simulink model "motor_maxon_EC20flat_351006"  (R2026a)
settings: Solver=FixedStepDiscrete  StopTime=5  FixedStep=Ts_sim
InitFcn:
  | warning('off','physmod:simscape:engine:core:advancer_errors:fallback_solve')
model workspace (MAT data in the model file):
  B_motor = 3.66016133122e-07
  B_rotor = 2e-07
  B_turntable = 5e-06
  C_buck = 4.7e-05
  Dmax = 0.95
  Fsw = 50000
  I_max = 1.5
  J_body = 0.002
  J_flywheel = 2.34905654183e-05
  J_rotor = 5.1e-07
  K_A = 1
  Ki_current = 22242.4759874
  Ki_pos = 33476.7250761
  Ki_speed = 0.557062597018
  Kp_current = 2.66407057024
  Kp_pos = 13714.3486588
  Kp_speed = 0.0153460770528
  Kt_motor = 0.00882
  L_buck = 0.0001
  L_motor = 0.000424
  R_motor = 3.54
  T_brk_motor = 0.00028915488
  T_brk_turntable = 0.0012
  T_col_motor = 0.0002409624
  T_col_turntable = 0.001
  Ts_inner = 2.5e-05
  Ts_outer = 0.01
  Ts_sim = 2.5e-05
  Vin = 9
  f_pwm = 5000
  psi_m = 0.004
  slew_acc_max = 1.2
  slew_rate_max = 0.5
  w_bias = 0
  w_max = 3000
libraries: fl_lib x11, nesl_utility x6, slpidlib x3, ee_lib x2
settings Model: Creator=mulusoy  LastModifiedBy=tama
settings SimscapeCC: SimscapeNominalValues="[{\"value\":\"1\",\"unit\":\"A\"},{\"value\":\"1\",\"unit\":\"bar\"},{\"value\":\"1\",\"unit\":\"cm^2\"},{\"value\":\"1\",\"unit\":\"cm^3/s\"},{\"value\":\"1\",\"unit\":\"kJ/kg\"},{\"value\":\"1\",\"unit\":\"kW\"},{\"value\":\"1\",\"unit\":\"l\"},{\"value\":\"1\",\"unit\":\"N\"},{\"value\":\"1\",\"unit\":\"N*m\"},{\"value\":\"1\",\"unit\":\"V\"}]"  SimscapeLogType=none  SimscapeLogDataHistory=5000.0

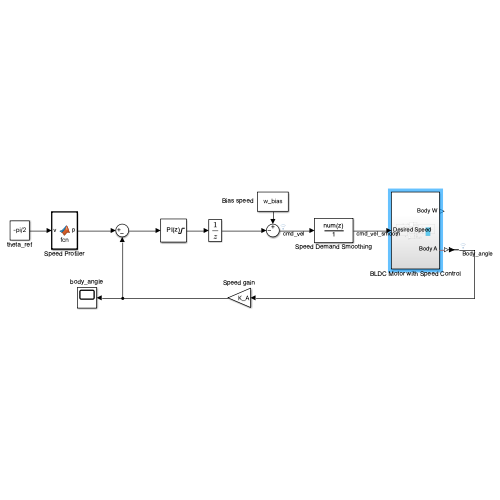
[thumbnail: Simulink's stored preview of the top-level diagram]
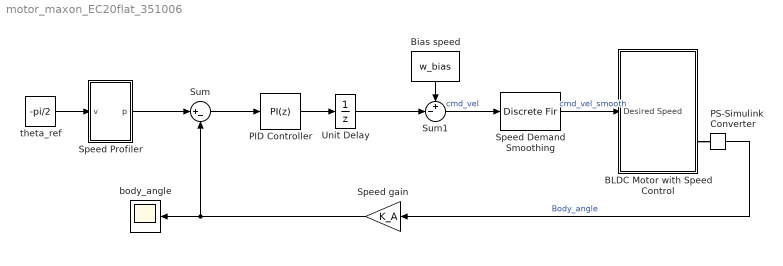
== system motor_maxon_EC20flat_351006 ==
  BLDC Motor with Speed Control : Subsystem
  Bias speed : Constant  Value=w_bias
  PID Controller : slpidlib/PID Controller  Controller=PI  Form=Parallel  TimeDomain=Discrete-time  UseExternalTs=off  SampleTime=0.01  IntegratorMethod=Forward Euler  FilterMethod=Forward Euler  ControllerParametersSource=internal  P=Kp_pos  I=Ki_pos  UseKiTs=off  D=0  UseExternalDerivativeSource=off  N=100  UseFilter=on  TunerSelectOption=Transfer Function Based (PID Tuner App)  InitialConditionSource=internal  InitialConditionForIntegrator=0  InitialConditionForFilter=0  DifferentiatorICPrevScaledInput=0  ExternalReset=none  TrackingMode=off  Kt=1  LimitOutput=on  SatLimitsSource=internal  UpperSaturationLimit=w_max  LowerSaturationLimit=-w_max  LinearizeAsGain=on  AntiWindupMode=clamping  Kb=1  LimitIntegrator=off  UpperIntegratorSaturationLimit=inf  LowerIntegratorSaturationLimit=-inf  POutMin=[]  POutMax=[]  IOutMin=[]  IOutMax=[]  DOutMin=[]  DOutMax=[]  NOutMin=[]  NOutMax=[]  SumOutMin=[]  SumOutMax=[]  SaturationOutMin=[]  SaturationOutMax=[]  PParamMin=[]  PParamMax=[]  IParamMin=[]  IParamMax=[]  DParamMin=[]  DParamMax=[]  NParamMin=[]  NParamMax=[]  KbParamMin=[]  KbParamMax=[]  KtParamMin=[]  KtParamMax=[]  KbOutMin=[]  KbOutMax=[]  KtOutMin=[]  KtOutMax=[]  IntegratorOutMin=[]  IntegratorOutMax=[]  FilterOutMin=[]  FilterOutMax=[]  SumI1OutMin=[]  SumI1OutMax=[]  SumI2OutMin=[]  SumI2OutMax=[]  SumI3OutMin=[]  SumI3OutMax=[]  SumI4OutMin=[]  SumI4OutMax=[]  SumDOutMin=[]  SumDOutMax=[]  DifferentiatorOutMin=[]  DifferentiatorOutMax=[]  FilterDiffOutCoefMin=[]  FilterDiffOutCoefMax=[]  ReciprocalOutMin=[]  ReciprocalOutMax=[]  SumDenOutMin=[]  SumDenOutMax=[]  SumNumOutMin=[]  SumNumOutMax=[]  DivideOutMin=[]  DivideOutMax=[]  UdiffTsProdOutMin=[]  UdiffTsProdOutMax=[]  NTsProdOutMin=[]  NTsProdOutMax=[]  UintegralTsProdOutMin=[]  UintegralTsProdOutMax=[]  UngainTsProdOutMin=[]  UngainTsProdOutMax=[]  ClampingZeroOutDataTypeStr=Inherit: Inherit via back propagation  ClampingZeroOutMin=[]  ClampingZeroOutMax=[]  FilterDenConstantOutDataTypeStr=Inherit: Inherit via back propagation  FilterDenConstantOutMin=[]  FilterDenConstantOutMax=[]  PCopyOutDataTypeStr=Inherit: Inherit via back propagation  PCopyOutMin=[]  PCopyOutMax=[]  NCopyOutDataTypeStr=Inherit: Inherit via back propagation  NCopyOutMin=[]  NCopyOutMax=[]  IntegratorContinuousStateAttributes=''  IntegratorStateMustResolveToSignalObject=off  IntegratorRTWStateStorageClass=Auto  FilterContinuousStateAttributes=''  FilterStateMustResolveToSignalObject=off  FilterRTWStateStorageClass=Auto  ParallelPVariant=InternalParameters  IdealPVariant=Disabled  IVariant=InternalParameters  DVariant=Disabled  IntegratorVariant=Discrete  SatVariant=Enabled  AWVariant=DiscClampingParallel  PCopyVariant=Disabled  TRVariant=Disabled  FdbkBlocksVariant=Forward  IdealPFdbkVariant=Disabled  SatFdbkVariant=Disabled  DerivativeFilterVariant=Disabled  NVariant=Disabled  NCopyVariant=Disabled_SignalSpec  FilterICVariant=Disabled  IntegratorICVariant=InternalICs  ExternalResetVariant=Disabled  TRSumVariant=Passthrough  SumFdbkVariant=Disabled  SumVariant=Sum_PI  TsampFilterVariant=InternalTs  TsampNgainVariant=Passthrough  TsampIntegralVariant=Disabled_SignalSpec  ExternalSaturationOutDataTypeStr=Inherit: Same as second input  DerivativeSourceVariant=Disabled  PreIntVariant=InternalPreInt
  PS-Simulink Converter : nesl_utility/PS-Simulink Converter  PhysicalDomain=network_engine_domain  SubClassName=ps_output  LeftPortType=input  RightPortType=output  PseudoPeriodic=off  Frequencies=[]  VectorFormat=inherit  Unit=inherit  AffineConversion=off
  Speed Demand Smoothing : DiscreteFir  Coefficients=ones(1,round(Ts_outer/Ts_inner))/round(Ts_outer/Ts_inner)  SampleTime=Ts_inner
  Speed Profiler : MATLAB Function  TreatAsAtomicUnit=on  SystemSampleTime=Ts_outer
  Speed gain : Gain  Gain=K_A
  Sum : Sum  Inputs=|+-
  Sum1 : Sum  Inputs=+-|
  Unit Delay : UnitDelay  SampleTime=-1
  body_angle : Scope
      settings: ActiveDisplayYMinimum=-1.7754175161910279  ActiveDisplayYMaximum=0.19726861291011416  DataLoggingVariableName=ScopeData3
  theta_ref : Constant  Value=-pi/2
  wires:
  PID Controller/1 -> Unit Delay/1
  theta_ref/1 -> Speed Profiler/1(v)
  Sum/1 -> PID Controller/1
  Speed gain/1 -> Sum/2, body_angle/1
  Bias speed/1 -> Sum1/1
  Unit Delay/1 -> Sum1/2
  Speed Profiler/1(p) -> Sum/1
  Speed Demand Smoothing/1 -> BLDC Motor with Speed Control/1(Desired Speed)  "cmd_vel_smooth"
  Sum1/1 -> Speed Demand Smoothing/1  "cmd_vel"
  PS-Simulink Converter/1 -> Speed gain/1  "Body_angle"
  connections:
  BLDC Motor with Speed Control/RConn2 -- PS-Simulink Converter/LConn1

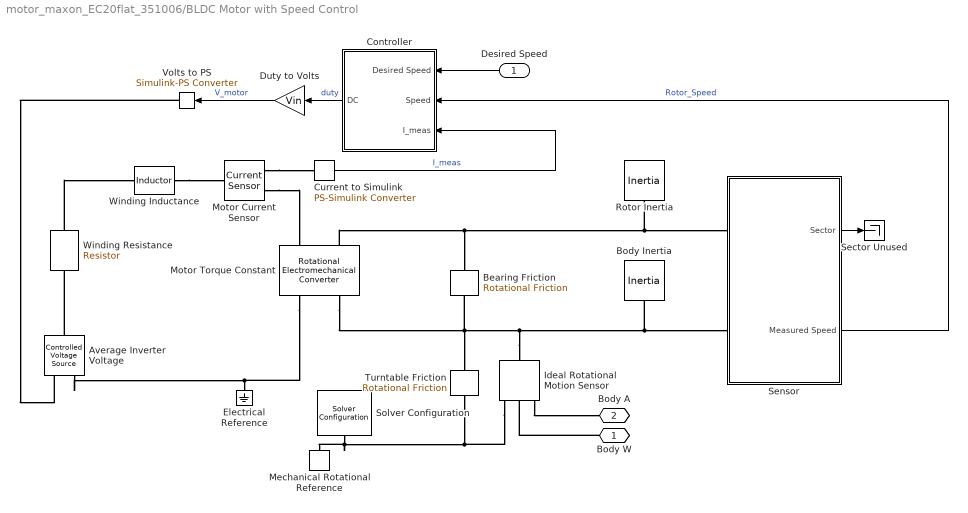
== system motor_maxon_EC20flat_351006/BLDC Motor with Speed Control ==
  Desired Speed : Inport
  Average Inverter Voltage : fl_lib/Electrical/Electrical Sources/Controlled Voltage Source
  Bearing Friction : fl_lib/Mechanical/Rotational Elements/Rotational Friction  brkwy_trq=T_brk_motor N*m  brkwy_vel=0.1 rad/s  Col_trq=T_col_motor N*m  visc_coef=B_motor N*m*s/rad  w_specify=off  w_priority=None  w=0 rad/s  w_nominal_specify=off  w_nominal_value=1  w_nominal_unit=rad/s  t_specify=off  t_priority=None  t=0 N*m  t_nominal_specify=off  t_nominal_value=1  t_nominal_unit=N*m
  Body Inertia : fl_lib/Mechanical/Rotational Elements/Inertia  inertia=J_body kg*m^2  num_ports=foundation.enum.numPorts2.one  w_specify=on  w_priority=High  w=0 rad/s  w_nominal_specify=off  w_nominal_value=1  w_nominal_unit=rad/s  t_specify=off  t_priority=None  t=0 N*m  t_nominal_specify=off  t_nominal_value=1  t_nominal_unit=N*m
  Controller : Subsystem
  Current to Simulink : nesl_utility/PS-Simulink Converter  PhysicalDomain=network_engine_domain  SubClassName=ps_output  LeftPortType=input  RightPortType=output  PseudoPeriodic=off  Frequencies=[]  VectorFormat=inherit  Unit=inherit  AffineConversion=off
  Duty to Volts : Gain  Gain=Vin
  Electrical Reference : fl_lib/Electrical/Electrical Elements/Electrical Reference
  Ideal Rotational Motion Sensor : fl_lib/Mechanical/Mechanical Sensors/Ideal Rotational Motion Sensor  reference=foundation.enum.MeasurementReference.difference  acceleration_port=false  velocity_port=true  position_port=true  wrap_angle=false  offset=0 rad
  Mechanical Rotational Reference : fl_lib/Mechanical/Rotational Elements/Mechanical Rotational Reference
  Motor Current Sensor : fl_lib/Electrical/Electrical Sensors/Current Sensor
  Motor Torque Constant : fl_lib/Electrical/Electrical Elements/Rotational Electromechanical Converter  K=Kt_motor V*s/rad  i_specify=off  i_priority=None  i=0 A  i_nominal_specify=off  i_nominal_value=1  i_nominal_unit=A  v_specify=off  v_priority=None  v=0 V  v_nominal_specify=off  v_nominal_value=1  v_nominal_unit=V  t_specify=off  t_priority=None  t=0 N*m  t_nominal_specify=off  t_nominal_value=1  t_nominal_unit=N*m  w_specify=off  w_priority=None  w=0 rad/s  w_nominal_specify=off  w_nominal_value=1  w_nominal_unit=rad/s
  Rotor Inertia : fl_lib/Mechanical/Rotational Elements/Inertia  inertia=J_flywheel + J_rotor kg*m^2  num_ports=foundation.enum.numPorts2.one  w_specify=on  w_priority=High  w=w_bias rpm  w_nominal_specify=off  w_nominal_value=1  w_nominal_unit=rad/s  t_specify=off  t_priority=None  t=0 N*m  t_nominal_specify=off  t_nominal_value=1  t_nominal_unit=N*m
  Sector Unused : Terminator
  Sensor : Subsystem
  Solver Configuration : nesl_utility/Solver Configuration  PhysicalDomain=network_engine_domain  SubClassName=solver  LeftPortType=input  RightPortType=generic  Tones=[]  Harmonics=[]  SimulateNoise=off  Profile=off  UseLocalSampling=off  EnableSwitchedLinearOptims=on  FrequencyDomain=off  UseCCode=off  RelTol=0.001  AbsTol=1e-06  MinStep=1e-09  ToWorkspace=off  RevertToSquareIcSolve=off  NumHomotopyIterations=100  PhasorMode=off  PhasorModeNumHarmonics=1  ConsistencySolver=NEWTON_FTOL  CanonicalOrdering=UNORDERED  OptimizeIntermediates=UNOPTIMIZED  IndexReductionMethod=DerivativeReplacement  DoDC=off  ResidualTolerance=1e-09  ConsistencyTolSource=GLOBAL  ConsistencyAbsTol=0.001  ConsistencyRelTol=0.001  ConsistencyTolFactor=0.001  UseLocalSolver=on  LocalSolverChoice=NE_BACKWARD_EULER_ADVANCER  ResolveIndetEquations=on  FunctionEvalNumThread=1  LocalSolverSampleTime=Ts_sim  DoFixedCost=on  MaxNonlinIter=4  MaxModeIter=2  ComputeImpulses=off  ImpulseIterations=2  LinearAlgebra=auto  LinearAlgebraNumThread=0  EquationFormulation=NE_TIME_EF  DelaysMemoryBudget=1024  AutomaticFiltering=off  FilteringTimeConstant=0.001  PartitionStorageMethod=AS_NEEDED  PartitionMemoryBudget=1024  PartitionMethod=ROBUST  MultibodyUseLocalSolver=off  MultibodyLocalSolverChoice=ODE1  MultibodyLocalSolverSampleTime=0.001
  Turntable Friction : fl_lib/Mechanical/Rotational Elements/Rotational Friction  brkwy_trq=T_brk_turntable N*m  brkwy_vel=0.1 rad/s  Col_trq=T_col_turntable N*m  visc_coef=B_turntable N*m*s/rad  w_specify=off  w_priority=None  w=0 rad/s  w_nominal_specify=off  w_nominal_value=1  w_nominal_unit=rad/s  t_specify=off  t_priority=None  t=0 N*m  t_nominal_specify=off  t_nominal_value=1  t_nominal_unit=N*m
  Volts to PS : nesl_utility/Simulink-PS Converter  PhysicalDomain=network_engine_domain  SubClassName=ps_input  LeftPortType=input  RightPortType=output  PseudoPeriodic=off  Frequencies=[]  NoiseDistribution=none  NoiseParameters=[]  Unit=1  AffineConversion=off  FilteringAndDerivatives=provide  SimscapeFilterOrder=1  InputFilterTimeConstant=0.001  UdotUserProvided=0
  Winding Inductance : ee_lib/Passive/Inductor  l=L_motor H  enable_L_tol=ee.enum.toleranceApplication.none  L_tol=20  tol_distribution=ee.enum.toleranceDistribution.uniform  nSigma=4  r=0 Ohm  g=1e-9 1/Ohm  enable_operating_limits=ee.enum.enable.no  operating_limit_action=ee.enum.passive.reportOpLim.warn  max_working_current=1 A  power_rating=1 W  i_L_specify=off  i_L_priority=High  i_L=0 A  i_L_nominal_specify=off  i_L_nominal_value=1  i_L_nominal_unit=A
  Winding Resistance : ee_lib/Passive/Resistor  R=R_motor Ohm  enable_R_tol=ee.enum.toleranceApplication.none  R_tol=5  tol_distribution=ee.enum.toleranceDistribution.uniform  nSigma=4  enable_operating_limits=ee.enum.enable.no  operating_limit_action=ee.enum.passive.reportOpLim.warn  power_rating=1 W  max_working_voltage=100 V  noise_mode=ee.enum.sources.noise.Disabled  Tdevice=25 degC  sample_time=1e-3 s  repeatability=ee.enum.ic.repeatability.notRepeatable  user_seed=0  auto_seed=3499211588  power_derating_T1=70 degC  power_derating_T2=155 degC  operating_temperature_range_vec=[-50, 150] degC  alpha=3.93e-3 1/K  Tmeas=25 degC  thermal_mass=100 J/K  temperature_specify=off  temperature_priority=High  temperature=298.15 K  temperature_nominal_specify=off  temperature_nominal_value=1  temperature_nominal_unit=K
  Body W : PMIOPort  Side=Right
  Body A : PMIOPort  Port=2  Side=Right
  wires:
  Current to Simulink/1 -> Controller/3(I_meas)  "I_meas"
  Duty to Volts/1 -> Volts to PS/1  "V_motor"
  Controller/1(DC) -> Duty to Volts/1  "duty"
  Sensor/1(Sector) -> Sector Unused/1
  Sensor/2(Measured Speed) -> Controller/2(Speed)  "Rotor_Speed"
  Desired Speed/1 -> Controller/1(Desired Speed)
  connections:
  Ideal Rotational Motion Sensor/RConn1 -- Mechanical Rotational Reference/LConn1 -- Solver Configuration/RConn1 -- Turntable Friction/RConn1
  Body W/RConn1 -- Ideal Rotational Motion Sensor/RConn2
  Ideal Rotational Motion Sensor/RConn3 -- Body A/RConn1
  Motor Current Sensor/RConn1 -- Current to Simulink/LConn1
  Average Inverter Voltage/RConn2 -- Motor Torque Constant/RConn1 -- Electrical Reference/LConn1
  Motor Current Sensor/RConn2 -- Motor Torque Constant/LConn1
  Winding Inductance/RConn1 -- Motor Current Sensor/LConn1
  Winding Resistance/RConn1 -- Winding Inductance/LConn1
  Average Inverter Voltage/LConn1 -- Winding Resistance/LConn1
  Volts to PS/RConn1 -- Average Inverter Voltage/RConn1
  Ideal Rotational Motion Sensor/LConn1 -- Motor Torque Constant/RConn2 -- Bearing Friction/RConn1 -- Turntable Friction/LConn1 -- Sensor/LConn2 -- Body Inertia/LConn1
  Rotor Inertia/LConn1 -- Sensor/LConn1 -- Motor Torque Constant/LConn2 -- Bearing Friction/LConn1

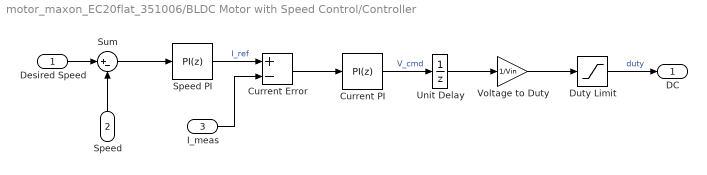
== system motor_maxon_EC20flat_351006/BLDC Motor with Speed Control/Controller ==
  Desired Speed : Inport
  Speed : Inport  Port=2
  I_meas : Inport  Port=3
  Current Error : Sum  Inputs=+-
  Current PI : slpidlib/PID Controller  Controller=PI  Form=Parallel  TimeDomain=Discrete-time  UseExternalTs=off  SampleTime=Ts_inner  IntegratorMethod=Forward Euler  FilterMethod=Forward Euler  ControllerParametersSource=internal  P=Kp_current  I=Ki_current  UseKiTs=off  D=0  UseExternalDerivativeSource=off  N=100  UseFilter=on  TunerSelectOption=Transfer Function Based (PID Tuner App)  InitialConditionSource=internal  InitialConditionForIntegrator=0  InitialConditionForFilter=0  DifferentiatorICPrevScaledInput=0  ExternalReset=none  TrackingMode=off  Kt=1  LimitOutput=on  SatLimitsSource=internal  UpperSaturationLimit=Dmax*Vin  LowerSaturationLimit=-Dmax*Vin  LinearizeAsGain=on  AntiWindupMode=clamping  Kb=1  LimitIntegrator=off  UpperIntegratorSaturationLimit=inf  LowerIntegratorSaturationLimit=-inf  POutMin=[]  POutMax=[]  IOutMin=[]  IOutMax=[]  DOutMin=[]  DOutMax=[]  NOutMin=[]  NOutMax=[]  SumOutMin=[]  SumOutMax=[]  SaturationOutMin=[]  SaturationOutMax=[]  PParamMin=[]  PParamMax=[]  IParamMin=[]  IParamMax=[]  DParamMin=[]  DParamMax=[]  NParamMin=[]  NParamMax=[]  KbParamMin=[]  KbParamMax=[]  KtParamMin=[]  KtParamMax=[]  KbOutMin=[]  KbOutMax=[]  KtOutMin=[]  KtOutMax=[]  IntegratorOutMin=[]  IntegratorOutMax=[]  FilterOutMin=[]  FilterOutMax=[]  SumI1OutMin=[]  SumI1OutMax=[]  SumI2OutMin=[]  SumI2OutMax=[]  SumI3OutMin=[]  SumI3OutMax=[]  SumI4OutMin=[]  SumI4OutMax=[]  SumDOutMin=[]  SumDOutMax=[]  DifferentiatorOutMin=[]  DifferentiatorOutMax=[]  FilterDiffOutCoefMin=[]  FilterDiffOutCoefMax=[]  ReciprocalOutMin=[]  ReciprocalOutMax=[]  SumDenOutMin=[]  SumDenOutMax=[]  SumNumOutMin=[]  SumNumOutMax=[]  DivideOutMin=[]  DivideOutMax=[]  UdiffTsProdOutMin=[]  UdiffTsProdOutMax=[]  NTsProdOutMin=[]  NTsProdOutMax=[]  UintegralTsProdOutMin=[]  UintegralTsProdOutMax=[]  UngainTsProdOutMin=[]  UngainTsProdOutMax=[]  ClampingZeroOutDataTypeStr=Inherit: Inherit via back propagation  ClampingZeroOutMin=[]  ClampingZeroOutMax=[]  FilterDenConstantOutDataTypeStr=Inherit: Inherit via back propagation  FilterDenConstantOutMin=[]  FilterDenConstantOutMax=[]  PCopyOutDataTypeStr=Inherit: Inherit via back propagation  PCopyOutMin=[]  PCopyOutMax=[]  NCopyOutDataTypeStr=Inherit: Inherit via back propagation  NCopyOutMin=[]  NCopyOutMax=[]  IntegratorContinuousStateAttributes=''  IntegratorStateMustResolveToSignalObject=off  IntegratorRTWStateStorageClass=Auto  FilterContinuousStateAttributes=''  FilterStateMustResolveToSignalObject=off  FilterRTWStateStorageClass=Auto  ParallelPVariant=InternalParameters  IdealPVariant=Disabled  IVariant=InternalParameters  DVariant=Disabled  IntegratorVariant=Discrete  SatVariant=Enabled  AWVariant=DiscClampingParallel  PCopyVariant=Disabled  TRVariant=Disabled  FdbkBlocksVariant=Forward  IdealPFdbkVariant=Disabled  SatFdbkVariant=Disabled  DerivativeFilterVariant=Disabled  NVariant=Disabled  NCopyVariant=Disabled_SignalSpec  FilterICVariant=Disabled  IntegratorICVariant=InternalICs  ExternalResetVariant=Disabled  TRSumVariant=Passthrough  SumFdbkVariant=Disabled  SumVariant=Sum_PI  TsampFilterVariant=InternalTs  TsampNgainVariant=Passthrough  TsampIntegralVariant=Disabled_SignalSpec  ExternalSaturationOutDataTypeStr=Inherit: Same as second input  DerivativeSourceVariant=Disabled  PreIntVariant=InternalPreInt
  Duty Limit : Saturate  UpperLimit=Dmax  LowerLimit=-Dmax
  Speed PI : slpidlib/PID Controller  Controller=PI  Form=Parallel  TimeDomain=Discrete-time  UseExternalTs=off  SampleTime=Ts_inner  IntegratorMethod=Forward Euler  FilterMethod=Forward Euler  ControllerParametersSource=internal  P=Kp_speed  I=Ki_speed  UseKiTs=off  D=0  UseExternalDerivativeSource=off  N=100  UseFilter=on  TunerSelectOption=Transfer Function Based (PID Tuner App)  InitialConditionSource=internal  InitialConditionForIntegrator=0  InitialConditionForFilter=0  DifferentiatorICPrevScaledInput=0  ExternalReset=none  TrackingMode=off  Kt=1  LimitOutput=on  SatLimitsSource=internal  UpperSaturationLimit=I_max  LowerSaturationLimit=-I_max  LinearizeAsGain=on  AntiWindupMode=clamping  Kb=1  LimitIntegrator=off  UpperIntegratorSaturationLimit=inf  LowerIntegratorSaturationLimit=-inf  POutMin=[]  POutMax=[]  IOutMin=[]  IOutMax=[]  DOutMin=[]  DOutMax=[]  NOutMin=[]  NOutMax=[]  SumOutMin=[]  SumOutMax=[]  SaturationOutMin=[]  SaturationOutMax=[]  PParamMin=[]  PParamMax=[]  IParamMin=[]  IParamMax=[]  DParamMin=[]  DParamMax=[]  NParamMin=[]  NParamMax=[]  KbParamMin=[]  KbParamMax=[]  KtParamMin=[]  KtParamMax=[]  KbOutMin=[]  KbOutMax=[]  KtOutMin=[]  KtOutMax=[]  IntegratorOutMin=[]  IntegratorOutMax=[]  FilterOutMin=[]  FilterOutMax=[]  SumI1OutMin=[]  SumI1OutMax=[]  SumI2OutMin=[]  SumI2OutMax=[]  SumI3OutMin=[]  SumI3OutMax=[]  SumI4OutMin=[]  SumI4OutMax=[]  SumDOutMin=[]  SumDOutMax=[]  DifferentiatorOutMin=[]  DifferentiatorOutMax=[]  FilterDiffOutCoefMin=[]  FilterDiffOutCoefMax=[]  ReciprocalOutMin=[]  ReciprocalOutMax=[]  SumDenOutMin=[]  SumDenOutMax=[]  SumNumOutMin=[]  SumNumOutMax=[]  DivideOutMin=[]  DivideOutMax=[]  UdiffTsProdOutMin=[]  UdiffTsProdOutMax=[]  NTsProdOutMin=[]  NTsProdOutMax=[]  UintegralTsProdOutMin=[]  UintegralTsProdOutMax=[]  UngainTsProdOutMin=[]  UngainTsProdOutMax=[]  ClampingZeroOutDataTypeStr=Inherit: Inherit via back propagation  ClampingZeroOutMin=[]  ClampingZeroOutMax=[]  FilterDenConstantOutDataTypeStr=Inherit: Inherit via back propagation  FilterDenConstantOutMin=[]  FilterDenConstantOutMax=[]  PCopyOutDataTypeStr=Inherit: Inherit via back propagation  PCopyOutMin=[]  PCopyOutMax=[]  NCopyOutDataTypeStr=Inherit: Inherit via back propagation  NCopyOutMin=[]  NCopyOutMax=[]  IntegratorContinuousStateAttributes=''  IntegratorStateMustResolveToSignalObject=off  IntegratorRTWStateStorageClass=Auto  FilterContinuousStateAttributes=''  FilterStateMustResolveToSignalObject=off  FilterRTWStateStorageClass=Auto  ParallelPVariant=InternalParameters  IdealPVariant=Disabled  IVariant=InternalParameters  DVariant=Disabled  IntegratorVariant=Discrete  SatVariant=Enabled  AWVariant=DiscClampingParallel  PCopyVariant=Disabled  TRVariant=Disabled  FdbkBlocksVariant=Forward  IdealPFdbkVariant=Disabled  SatFdbkVariant=Disabled  DerivativeFilterVariant=Disabled  NVariant=Disabled  NCopyVariant=Disabled_SignalSpec  FilterICVariant=Disabled  IntegratorICVariant=InternalICs  ExternalResetVariant=Disabled  TRSumVariant=Passthrough  SumFdbkVariant=Disabled  SumVariant=Sum_PI  TsampFilterVariant=InternalTs  TsampNgainVariant=Passthrough  TsampIntegralVariant=Disabled_SignalSpec  ExternalSaturationOutDataTypeStr=Inherit: Same as second input  DerivativeSourceVariant=Disabled  PreIntVariant=InternalPreInt
  Sum : Sum  Inputs=|+-
  Unit Delay : UnitDelay  SampleTime=-1
  Voltage to Duty : Gain  Gain=1/Vin
  DC : Outport
  wires:
  Speed/1 -> Sum/2
  Desired Speed/1 -> Sum/1
  Current PI/1 -> Unit Delay/1  "V_cmd"
  Current Error/1 -> Current PI/1
  I_meas/1 -> Current Error/2
  Speed PI/1 -> Current Error/1  "I_ref"
  Voltage to Duty/1 -> Duty Limit/1
  Sum/1 -> Speed PI/1
  Unit Delay/1 -> Voltage to Duty/1
  Duty Limit/1 -> DC/1  "duty"

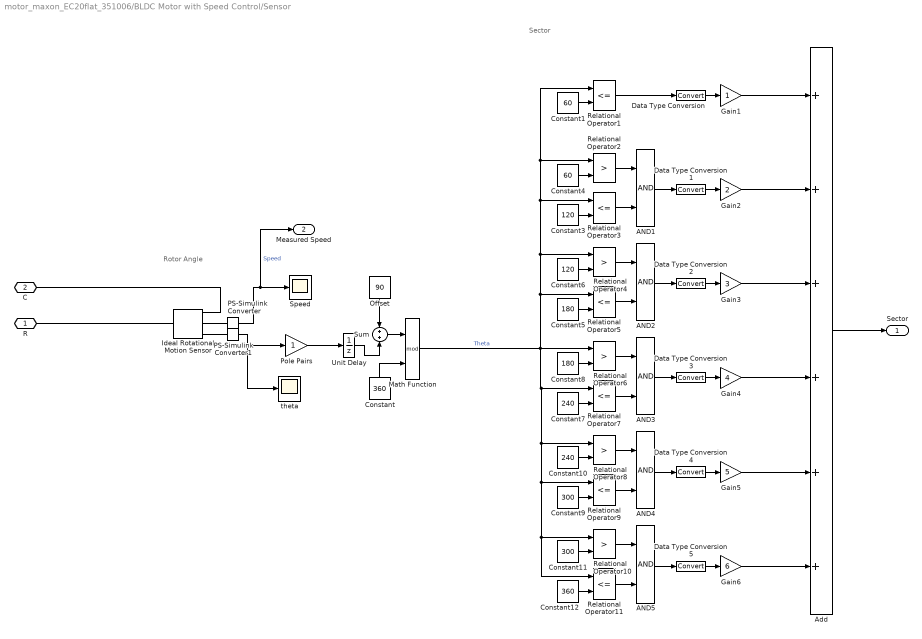
== system motor_maxon_EC20flat_351006/BLDC Motor with Speed Control/Sensor ==
  note: Rotor Angle
  note: Sector
  AND{1..5} (5 alike) : Logic  AllPortsSameDT=off  OutDataTypeStr=boolean
  Add : Sum  Inputs=6
  Constant : Constant  Value=360
  Constant1 : Constant  Value=60
  Constant10 : Constant  Value=240
  Constant11 : Constant  Value=300
  Constant12 : Constant  Value=360
  Constant3 : Constant  Value=120
  Constant4 : Constant  Value=60
  Constant5 : Constant  Value=180
  Constant6 : Constant  Value=120
  Constant7 : Constant  Value=240
  Constant8 : Constant  Value=180
  Constant9 : Constant  Value=300
  Data Type Conversion{,1..5} (6 alike) : DataTypeConversion  SaturateOnIntegerOverflow=off  RndMeth=Floor
  Gain1 : Gain
  Gain2 : Gain  Gain=2
  Gain3 : Gain  Gain=3
  Gain4 : Gain  Gain=4
  Gain5 : Gain  Gain=5
  Gain6 : Gain  Gain=6
  Ideal Rotational Motion Sensor : fl_lib/Mechanical/Mechanical Sensors/Ideal Rotational Motion Sensor  reference=foundation.enum.MeasurementReference.difference  acceleration_port=false  velocity_port=true  position_port=true  wrap_angle=false  offset=0 deg
  Math Function : Math  Operator=mod
  Offset : Constant  Value=90
  PS-Simulink Converter : nesl_utility/PS-Simulink Converter  PhysicalDomain=network_engine_domain  SubClassName=ps_output  LeftPortType=input  RightPortType=output  PseudoPeriodic=off  Frequencies=[]  VectorFormat=1-D array  Unit=rpm  AffineConversion=off
  PS-Simulink Converter1 : nesl_utility/PS-Simulink Converter  PhysicalDomain=network_engine_domain  SubClassName=ps_output  LeftPortType=input  RightPortType=output  PseudoPeriodic=off  Frequencies=[]  VectorFormat=1-D array  Unit=deg  AffineConversion=off
  Pole Pairs : Gain
  Relational Operator{1,3,5,7,9,11} (6 alike) : RelationalOperator  Operator=<=  OutDataTypeStr=boolean  RndMeth=Simplest  InputSameDT=off
  Relational Operator{2,4,6,8,10} (5 alike) : RelationalOperator  Operator=>  OutDataTypeStr=boolean  RndMeth=Simplest  InputSameDT=off
  Speed : Scope
      settings: ActiveDisplayYMinimum=-51.95479  ActiveDisplayYMaximum=223.68655  DataLoggingVariableName=theta
  Sum : Sum  Inputs=+|+
  Unit Delay : UnitDelay  SampleTime=-1
  theta : Scope
      settings: ActiveDisplayYMinimum=-1  ActiveDisplayYMaximum=1  DataLoggingVariableName=ScopeData2
  R : PMIOPort  Side=Left
  C : PMIOPort  Port=2  Side=Left
  Sector : Outport
  Measured Speed : Outport  Port=2
  wires:
  Add/1 -> Sector/1
  Gain6/1 -> Add/6
  Gain5/1 -> Add/5
  Gain4/1 -> Add/4
  Gain3/1 -> Add/3
  Gain2/1 -> Add/2
  Gain1/1 -> Add/1
  Relational Operator5/1 -> AND2/2
  Relational Operator10/1 -> AND5/1
  AND1/1 -> Data Type Conversion1/1
  Constant11/1 -> Relational Operator10/2
  AND5/1 -> Data Type Conversion5/1
  Constant12/1 -> Relational Operator11/2
  Data Type Conversion/1 -> Gain1/1
  AND2/1 -> Data Type Conversion2/1
  Relational Operator1/1 -> Data Type Conversion/1
  Data Type Conversion2/1 -> Gain3/1
  Data Type Conversion1/1 -> Gain2/1
  Data Type Conversion5/1 -> Gain6/1
  AND3/1 -> Data Type Conversion3/1
  Constant8/1 -> Relational Operator6/2
  Constant7/1 -> Relational Operator7/2
  Relational Operator6/1 -> AND3/1
  Data Type Conversion4/1 -> Gain5/1
  Relational Operator2/1 -> AND1/1
  AND4/1 -> Data Type Conversion4/1
  Relational Operator9/1 -> AND4/2
  Constant5/1 -> Relational Operator5/2
  Relational Operator3/1 -> AND1/2
  Constant3/1 -> Relational Operator3/2
  Relational Operator7/1 -> AND3/2
  Relational Operator4/1 -> AND2/1
  Constant4/1 -> Relational Operator2/2
  Constant1/1 -> Relational Operator1/2
  Data Type Conversion3/1 -> Gain4/1
  Relational Operator8/1 -> AND4/1
  Constant10/1 -> Relational Operator8/2
  Constant6/1 -> Relational Operator4/2
  Constant9/1 -> Relational Operator9/2
  Relational Operator11/1 -> AND5/2
  Math Function/1 -> Relational Operator6/1, Relational Operator1/1, Relational Operator2/1, Relational Operator3/1, Relational Operator4/1, Relational Operator5/1, Relational Operator7/1, Relational Operator8/1, Relational Operator10/1, Relational Operator11/1, Relational Operator9/1  "Theta"
  Pole Pairs/1 -> Unit Delay/1
  PS-Simulink Converter1/1 -> theta/1, Pole Pairs/1
  PS-Simulink Converter/1 -> Measured Speed/1, Speed/1  "Speed"
  Constant/1 -> Math Function/2
  Unit Delay/1 -> Sum/2
  Offset/1 -> Sum/1
  Sum/1 -> Math Function/1
  connections:
  Ideal Rotational Motion Sensor/LConn1 -- R/RConn1
  PS-Simulink Converter/LConn1 -- Ideal Rotational Motion Sensor/RConn2
  Ideal Rotational Motion Sensor/RConn1 -- C/RConn1
  Ideal Rotational Motion Sensor/RConn3 -- PS-Simulink Converter1/LConn1

== matlab function motor_maxon_EC20flat_351006/Speed Profiler ==
  data: v input; p output; slew_acc_max parameter; slew_rate_max parameter; Ts_outer parameter
function p = fcn(v, slew_acc_max, slew_rate_max, Ts_outer)
% Trapezoidal slew profile: moves the angle reference p towards the
% target v with body rate limited to slew_rate_max (rad/s) and body
% acceleration limited to slew_acc_max (rad/s^2). The target can change
% at any time; the profile replans from its current position and rate.

persistent pos rate
if isempty(pos)
    pos = 0;    % body starts at 0 rad
    rate = 0;
end

d = v - pos;

% Fastest rate that can still stop at the target, decelerating at
% slew_acc_max in discrete steps of Ts_outer
rateStop = slew_acc_max*(sqrt((Ts_outer/2)^2 + 2*abs(d)/slew_acc_max) - Ts_outer/2);
rateDes = sign(d)*min(slew_rate_max, rateStop);

% Move towards the desired rate without exceeding the acceleration limit
dRate = rateDes - rate;
rate = rate + max(-slew_acc_max*Ts_outer, min(slew_acc_max*Ts_outer, dRate));
pos = pos + rate*Ts_outer;

% Snap onto the target once there
if abs(v - pos) < 1e-6 && abs(rate) < slew_acc_max*Ts_outer
    pos = v;
    rate = 0;
end

p = pos;
